simulink subsystem "PowerSystemRefAeronomie"  (R2024b)
settings: Solver=VariableStepAuto  StartTime=0.0  StopTime=10.0  RelTol=1e-3
undefined symbols (not defined in the file or in its folder): ess, mot, powerplant, propel, pxf_diagram_options, SimIn, tc
libraries: simulink x2, slpidlib x1, matrix_library x1
(part 3 of 3)

== system PowerSystemRefAeronomie/ess (battery)/ctrl/ess_ctrl_pngv_map_anl_PI_cstr/PI controller for maximal charge power and current1/PI Ratio Calculator (curr) 1 ==
  note: %deviation
  ess pwr : Inport
  pwr max cont : Inport  Port=2
  Add1 : Sum  Inputs=-+
  Integrator1 : Integrator  InitialCondition=ess.plant.init.ul_curr_dis  LimitOutput=on  UpperSaturationLimit=ess.plant.init.ul_curr_dis  LowerSaturationLimit=ess.plant.init.ll_curr_dis
  Ki_pwr : Gain  Gain=ess.plant.init.Ki_pwr_chg  SaturateOnIntegerOverflow=on  OutDataTypeStr=Inherit: Same as input  ParamDataTypeStr=Inherit: Same as input
  Saturation1 : Saturate  UpperLimit=1  LowerLimit=0
  non-zero division1 : Subsystem
      mask Display: disp('divider')
  pwr ratio : Outport
  wires:
  Add1/1 -> non-zero division1/1(In1)
  non-zero division1/1(Out1) -> Ki_pwr/1
  Ki_pwr/1 -> Integrator1/1
  Integrator1/1 -> Saturation1/1
  ess pwr/1 -> Add1/1
  Saturation1/1 -> pwr ratio/1
  pwr max cont/1 -> Add1/2, non-zero division1/2(In2)

== system PowerSystemRefAeronomie/ess (battery)/ctrl/ess_ctrl_pngv_map_anl_PI_cstr/PI controller for maximal discharge power and current1/PI Ratio Calculator (curr)  ==
  note: %deviation
  ess curr : Inport
  curr max cont : Inport  Port=2
  Add1 : Sum  Inputs=-+
  Integrator1 : Integrator  InitialCondition=ess.plant.init.ul_curr_dis  LimitOutput=on  UpperSaturationLimit=ess.plant.init.ul_curr_dis  LowerSaturationLimit=ess.plant.init.ll_curr_dis
  Ki_curr : Gain  Gain=ess.plant.init.Ki_curr_dis  SaturateOnIntegerOverflow=on  OutDataTypeStr=Inherit: Same as input  ParamDataTypeStr=Inherit: Same as input
  Saturation1 : Saturate  UpperLimit=1  LowerLimit=0
  non-zero division1 : Subsystem
      mask Display: disp('divider')
  Current ratio : Outport
  wires:
  curr max cont/1 -> non-zero division1/2(In2), Add1/2
  Saturation1/1 -> Current ratio/1
  ess curr/1 -> Add1/1
  Integrator1/1 -> Saturation1/1
  Ki_curr/1 -> Integrator1/1
  non-zero division1/1(Out1) -> Ki_curr/1
  Add1/1 -> non-zero division1/1(In1)

== system PowerSystemRefAeronomie/ess (battery)/ctrl/ess_ctrl_pngv_map_anl_PI_cstr/PI controller for maximal discharge power and current1/PI Ratio Calculator (curr) 1 ==
  note: %deviation
  ess pwr : Inport
  pwr max cont : Inport  Port=2
  Add1 : Sum  Inputs=-+
  Integrator1 : Integrator  InitialCondition=ess.plant.init.ul_curr_dis  LimitOutput=on  UpperSaturationLimit=ess.plant.init.ul_curr_dis  LowerSaturationLimit=ess.plant.init.ll_curr_dis
  Ki_pwr : Gain  Gain=ess.plant.init.Ki_pwr_dis  SaturateOnIntegerOverflow=on  OutDataTypeStr=Inherit: Same as input  ParamDataTypeStr=Inherit: Same as input
  Saturation1 : Saturate  UpperLimit=1  LowerLimit=0
  non-zero division1 : Subsystem
      mask Display: disp('divider')
  pwr ratio : Outport
  wires:
  Add1/1 -> non-zero division1/1(In1)
  non-zero division1/1(Out1) -> Ki_pwr/1
  Ki_pwr/1 -> Integrator1/1
  Integrator1/1 -> Saturation1/1
  ess pwr/1 -> Add1/1
  Saturation1/1 -> pwr ratio/1
  pwr max cont/1 -> Add1/2, non-zero division1/2(In2)

== system PowerSystemRefAeronomie/ess (battery)/plant/ess_plant_pngv_map_anl_PI_cstr/ess_cell/current polarization ==
  ess soc : Inport
  ess curr : Inport  Port=2
  Integrator : Integrator
  Product1 : Product  Inputs=*/  InputSameDT=on  SaturateOnIntegerOverflow=on  OutDataTypeStr=Inherit: Same as first input
  Sum1 : Sum  Inputs=+-  InputSameDT=on  SaturateOnIntegerOverflow=on  OutDataTypeStr=Inherit: Same as first input
  Time Constant : Lookup  InputValues=ess.plant.init.tau1.idx1_soc  Table=ess.plant.init.tau1.map
  ess_cell_curr_polar1 : Outport
  wires:
  Time Constant/1 -> Product1/2
  Product1/1 -> Integrator/1
  ess soc/1 -> Time Constant/1
  ess curr/1 -> Sum1/1
  Sum1/1 -> Product1/1
  Integrator/1 -> Sum1/2, ess_cell_curr_polar1/1

== system PowerSystemRefAeronomie/ess (battery)/plant/ess_plant_pngv_map_anl_PI_cstr/ess_cell/current polarization1 ==
  ess soc : Inport
  ess curr : Inport  Port=2
  Integrator : Integrator
  Product1 : Product  Inputs=*/  InputSameDT=on  SaturateOnIntegerOverflow=on  OutDataTypeStr=Inherit: Same as first input
  Sum1 : Sum  Inputs=+-  InputSameDT=on  SaturateOnIntegerOverflow=on  OutDataTypeStr=Inherit: Same as first input
  Time Constant : Lookup  InputValues=ess.plant.init.tau2.idx1_soc  Table=ess.plant.init.tau2.map
  ess_cell_curr_polar2 : Outport
  wires:
  Integrator/1 -> ess_cell_curr_polar2/1, Sum1/2
  Sum1/1 -> Product1/1
  ess curr/1 -> Sum1/1
  ess soc/1 -> Time Constant/1
  Product1/1 -> Integrator/1
  Time Constant/1 -> Product1/2

== system PowerSystemRefAeronomie/ess (battery)/plant/ess_plant_pngv_map_anl_PI_cstr/ess_cell/ess_soc_calculation ==
  cell_curr : Inport
  (sec->hrs) : Gain  Gain=1/3600  SaturateOnIntegerOverflow=on  OutDataTypeStr=Inherit: Same as input  ParamDataTypeStr=Inherit: Same as input
  (sec->hrs)1 : Gain  Gain=-1  SaturateOnIntegerOverflow=on  OutDataTypeStr=Inherit: Same as input  ParamDataTypeStr=Inherit: Same as input
  0 <= SOC <= 1 : Saturate  UpperLimit=1  LowerLimit=0
  1\ess.plant.init.cap : Gain  Gain=1/ess.plant.init.cap  SaturateOnIntegerOverflow=on  OutDataTypeStr=Inherit: Same as input  ParamDataTypeStr=Inherit: Same as input
  Integrator : Integrator  InitialCondition=ess.plant.init.soc_init
  ess_soc : Outport
  wires:
  (sec->hrs)/1 -> 1\ess.plant.init.cap/1
  0 <= SOC <= 1/1 -> ess_soc/1
  Integrator/1 -> 0 <= SOC <= 1/1
  (sec->hrs)1/1 -> Integrator/1
  1\ess.plant.init.cap/1 -> (sec->hrs)1/1
  cell_curr/1 -> (sec->hrs)/1

== system PowerSystemRefAeronomie/ess (battery)/plant/ess_plant_pngv_map_anl_PI_cstr/ess_cell/voltage calculation ==
  absolute SOC : Inport
  ess_cell_curr : Inport  Port=2
  ess_cell_curr_pol1 : Inport  Port=3
  ess_cell_curr_plo2 : Inport  Port=4
  Ohmic resist : Lookup  InputValues=ess.plant.init.rint.idx1_soc  Table=ess.plant.init.rint.map
  "Polarization resist 2 " : Lookup  InputValues=ess.plant.init.rpol2.idx1_soc  Table=ess.plant.init.rpol2.map
  Polarization resist2 : Lookup  InputValues=ess.plant.init.rpol1.idx1_soc  Table=ess.plant.init.rpol1.map
  Product1 : Product  InputSameDT=on  SaturateOnIntegerOverflow=on  OutDataTypeStr=Inherit: Same as first input
  Product2 : Product  InputSameDT=on  SaturateOnIntegerOverflow=on  OutDataTypeStr=Inherit: Same as first input
  Product3 : Product  InputSameDT=on  SaturateOnIntegerOverflow=on  OutDataTypeStr=Inherit: Same as first input
  Saturation : Saturate  UpperLimit=inf  LowerLimit=ess.plant.init.volt_min_burst
  Sum2 : Sum  Inputs=+---  InputSameDT=on  SaturateOnIntegerOverflow=on  OutDataTypeStr=Inherit: Same as first input
  Voc : Lookup  InputValues=ess.plant.init.voc.idx1_soc  Table=ess.plant.init.voc.map
  ess_cell_volt : Outport
  ess_cell_voc : Outport  Port=2
  ess_cell_rint : Outport  Port=3
  ess_cell_rpol1 : Outport  Port=4
  ess_cell_rpol2 : Outport  Port=5
  wires:
  Saturation/1 -> ess_cell_volt/1
  "Polarization resist 2 "/1 -> ess_cell_rpol2/1, Product3/2  "ess_rpol2_simu"
  ess_cell_curr_plo2/1 -> Product3/1
  Product3/1 -> Sum2/4
  Product2/1 -> Sum2/3
  Polarization resist2/1 -> ess_cell_rpol1/1, Product2/2  "ess_rpol1_simu"
  ess_cell_curr_pol1/1 -> Product2/1
  Product1/1 -> Sum2/2
  absolute SOC/1 -> Voc/1, Ohmic resist/1, Polarization resist2/1, "Polarization resist 2 "/1
  Voc/1 -> ess_cell_voc/1, Sum2/1  "ess_voc_simu"
  ess_cell_curr/1 -> Product1/1
  Ohmic resist/1 -> ess_cell_rint/1, Product1/2  "ess_rint_simu"
  Sum2/1 -> Saturation/1

== system PowerSystemRefAeronomie/mot/ctrl/cmd/mot_ctrl_cmd_map_Pelec_funTW_volt_in/Subsystem2 ==
  In1 : Inport
  In2 : Inport  Port=2
  Fcn : Fcn  Expr=u[1]/(u[2]+eps)*(u[2]!=0)
  Mux : Mux  Inputs=2
  Out1 : Outport
  wires:
  In2/1 -> Mux/2
  Fcn/1 -> Out1/1
  In1/1 -> Mux/1
  Mux/1 -> Fcn/1

== system PowerSystemRefAeronomie/mot/ctrl/cmd/mot_ctrl_cmd_map_Pelec_funTW_volt_in/avoid zero output ==
  In1 : Inport
  Constant : Constant  Value=eps
  Switch1 : Switch  Criteria=u2 ~= 0  SaturateOnIntegerOverflow=off  InputSameDT=off
  Out1 : Outport
  wires:
  In1/1 -> Switch1/2, Switch1/1
  Constant/1 -> Switch1/3
  Switch1/1 -> Out1/1

== system PowerSystemRefAeronomie/mot/ctrl/cstr/mot_ctrl_cstr_map_Pelec_funTW_volt_in/Continuous torque - Prop ==
  input x : Inport
  map : Lookup  InputValues=x  Table=map
  map limits on x : Saturate  UpperLimit=max(x)  LowerLimit=min(x)
  output : Outport
  wires:
  map limits on x/1 -> map/1
  map/1 -> output/1
  input x/1 -> map limits on x/1

== system PowerSystemRefAeronomie/mot/ctrl/cstr/mot_ctrl_cstr_map_Pelec_funTW_volt_in/Continuous torque _regen ==
  input x : Inport
  map : Lookup  InputValues=x  Table=map
  map limits on x : Saturate  UpperLimit=max(x)  LowerLimit=min(x)
  output : Outport
  wires:
  map limits on x/1 -> map/1
  map/1 -> output/1
  input x/1 -> map limits on x/1

== system PowerSystemRefAeronomie/mot/ctrl/cstr/mot_ctrl_cstr_map_Pelec_funTW_volt_in/Peak torque - Prop ==
  input x : Inport
  map : Lookup  InputValues=x  Table=map
  map limits on x : Saturate  UpperLimit=max(x)  LowerLimit=min(x)
  output : Outport
  wires:
  map limits on x/1 -> map/1
  map/1 -> output/1
  input x/1 -> map limits on x/1

== system PowerSystemRefAeronomie/mot/ctrl/cstr/mot_ctrl_cstr_map_Pelec_funTW_volt_in/Peak torque _regen ==
  input x : Inport
  map : Lookup  InputValues=x  Table=map
  map limits on x : Saturate  UpperLimit=max(x)  LowerLimit=min(x)
  output : Outport
  wires:
  map limits on x/1 -> map/1
  map/1 -> output/1
  input x/1 -> map limits on x/1

== system PowerSystemRefAeronomie/mot/ctrl/dmd/mot_ctrl_dmd_uas/Determine_Required_Motor_RPS ==
  Prop_D : Inport
  rho : Inport  Port=2
  P : Inport  Port=3
  Vtas : Inport  Port=4
  Algebraic Constraint1 : AlgebraicConstraint  InitialGuess=propel.ctrl.init.rps
  CP : Polyval  Coefs=powerplant.propel.init.CPpoly
  Fcn1 : Fcn  Expr=u(4)*u(5)^3 - u(3)/(u(2)*u(1)^5)
  Mux1 : Mux  Inputs=5
  Product : Product  Inputs=*//
  RPS_req : Outport  VectorParamsAs1DForOutWhenUnconnected=off
  wires:
  Vtas/1 -> Product/1
  Prop_D/1 -> Mux1/1, Product/2
  CP/1 -> Mux1/4
  Product/1 -> CP/1
  P/1 -> Mux1/3
  Mux1/1 -> Fcn1/1
  Fcn1/1 -> Algebraic Constraint1/1
  Algebraic Constraint1/1 -> RPS_req/1, Mux1/5, Product/3  "RPS_req"
  rho/1 -> Mux1/2

== system PowerSystemRefAeronomie/mot/ctrl/dmd/parameter_selection/Subsystem ==
  <EngineCmd> : Inport
  <Density> : Inport  Port=2
  Vtas : Inport  Port=3
  CP : Polyval  Coefs=powerplant.propel.init.CPpoly
  Constant8 : Constant  Value=mot.propel.plant.init.propD
  Fcn : Fcn  Expr=u(1)*u(2)*u(3)^3*u(4)^5
  Mux : Mux
  Normalize : Gain  Gain=1/mot.propel.plant.init.Pmax
  Product : Product  Inputs=*//
  Selector : Selector  InputPortWidth=9  IndexOptions=Index vector (dialog)  Indices=9  OutputSizes=1
  Transfer Fcn : TransferFcn  Numerator=1  Denominator=[0.01 1]
  rad/s to RPS : Gain  Gain=1/(2*pi)
  EnginePwrCmd : Outport
  wires:
  Fcn/1 -> Normalize/1
  Transfer Fcn/1 -> EnginePwrCmd/1
  rad/s to RPS/1 -> Mux/3, Product/3
  Vtas/1 -> Product/1
  Normalize/1 -> Transfer Fcn/1
  Mux/1 -> Fcn/1
  Selector/1 -> rad/s to RPS/1
  <Density>/1 -> Mux/2
  CP/1 -> Mux/1
  <EngineCmd>/1 -> Selector/1
  Constant8/1 -> Mux/4, Product/2
  Product/1 -> CP/1

== system PowerSystemRefAeronomie/mot/plant/mot_plant_map_Pelec_funTW_volt_in/max torque /Cont trq max - Prop ==
  input x : Inport
  map : Lookup  InputValues=x  Table=map
  map limits on x : Saturate  UpperLimit=max(x)  LowerLimit=min(x)
  output : Outport
  wires:
  input x/1 -> map limits on x/1
  map/1 -> output/1
  map limits on x/1 -> map/1

== system PowerSystemRefAeronomie/mot/plant/mot_plant_map_Pelec_funTW_volt_in/max torque /Cont trq max - Regen ==
  input x : Inport
  map : Lookup  InputValues=x  Table=map
  map limits on x : Saturate  UpperLimit=max(x)  LowerLimit=min(x)
  output : Outport
  wires:
  map limits on x/1 -> map/1
  map/1 -> output/1
  input x/1 -> map limits on x/1

== system PowerSystemRefAeronomie/mot/plant/mot_plant_map_Pelec_funTW_volt_in/max torque /Heat index ==
  note: Heat index calculation
  note: to avoid spikes
      |  due to
      | div by zero
  cont torque : Inport
  torque : Inport  Port=2
  Abs : Abs
  Divide : Subsystem  mask(Divide){}
      mask Display: disp('Divide')
  Heat Energy Factor : Integrator  InitialCondition=-0.3  LimitOutput=on  UpperSaturationLimit=1  LowerSaturationLimit=-0.3
  Heating Constant : Gain  Gain=0.3/mot.plant.init.t_max_trq  SaturateOnIntegerOverflow=on  OutDataTypeStr=Inherit: Same as input  ParamDataTypeStr=Inherit: Same as input
  Saturation : Saturate  UpperLimit=1  LowerLimit=0
  Saturation1 : Saturate  UpperLimit=10  LowerLimit=0
  Sum : Sum  Inputs=+-  InputSameDT=on  SaturateOnIntegerOverflow=on  OutDataTypeStr=Inherit: Same as first input
  motor inertia (Nms^2\rad)5 : Constant
  Heat index : Outport
  wires:
  Saturation1/1 -> Sum/1
  torque/1 -> Divide/1(numerator)
  Heat Energy Factor/1 -> Saturation/1
  Heating Constant/1 -> Heat Energy Factor/1
  Sum/1 -> Heating Constant/1
  Divide/1(quotient) -> Abs/1
  motor inertia (Nms^2\rad)5/1 -> Sum/2
  Saturation/1 -> Heat index/1
  Abs/1 -> Saturation1/1
  cont torque/1 -> Divide/2(denominator)

== system PowerSystemRefAeronomie/mot/plant/mot_plant_map_Pelec_funTW_volt_in/max torque /Peak trq max - Prop ==
  input x : Inport
  map : Lookup  InputValues=x  Table=map
  map limits on x : Saturate  UpperLimit=max(x)  LowerLimit=min(x)
  output : Outport
  wires:
  map limits on x/1 -> map/1
  map/1 -> output/1
  input x/1 -> map limits on x/1

== system PowerSystemRefAeronomie/mot/plant/mot_plant_map_Pelec_funTW_volt_in/max torque /Peak trq max - Regen ==
  input x : Inport
  map : Lookup  InputValues=x  Table=map
  map limits on x : Saturate  UpperLimit=max(x)  LowerLimit=min(x)
  output : Outport
  wires:
  input x/1 -> map limits on x/1
  map/1 -> output/1
  map limits on x/1 -> map/1

== system PowerSystemRefAeronomie/propel/plant/propel_plant_uas/Total_Moment/Moment_due_to_eng_position ==
  Vec 1 : Inport
  Vec 2 : Inport  Port=2
  Mux : Mux  Inputs=2
  Mux1 : Mux  Inputs=3
  i axis : Fcn  Expr=u[6]*u[2] - u[5]*u[3]
  j axis : Fcn  Expr=u[4]*u[3] - u[6]*u[1]
  k axis : Fcn  Expr=u[5]*u[1] - u[4]*u[2]
  X Prod : Outport  VectorParamsAs1DForOutWhenUnconnected=off
  wires:
  Mux1/1 -> X Prod/1
  k axis/1 -> Mux1/3
  i axis/1 -> Mux1/1
  j axis/1 -> Mux1/2
  Mux/1 -> i axis/1, k axis/1, j axis/1
  Vec 1/1 -> Mux/1
  Vec 2/1 -> Mux/2

== system PowerSystemRefAeronomie/tc/plant/tc_plant_map_trqloss_funTW/Torque calculation/Blending (state dependent) ==
  Input : Inport
  Control (state) : Inport  Port=2
  Linear spline : Fcn  Expr=(u<xl)*yl + (xl<=u)*(u<xc)*((yc-yl)*(u-xl)/(xc-xl)+yl) + (xc<=u)*(u<xr)*((yc-yr)*(u-xr)/(xc-xr)+yr) + (xr<=u)*yr
  Product2 : Product  InputSameDT=on  SaturateOnIntegerOverflow=on  OutDataTypeStr=Inherit: Same as first input
  Output : Outport
  wires:
  Input/1 -> Product2/1
  Linear spline/1 -> Product2/2
  Product2/1 -> Output/1
  Control (state)/1 -> Linear spline/1

== system PowerSystemRefAeronomie/tc/plant/tc_plant_map_trqloss_funTW/Torque calculation/trq losses ==
  Rows : Inport
  Cols : Inport  Port=2
  Look-Up Table (2-D) : Lookup2D  RowIndex=x  ColumnIndex=y  Table=t
  Out1 : Outport
  wires:
  Look-Up Table (2-D)/1 -> Out1/1
  Cols/1 -> Look-Up Table (2-D)/2
  Rows/1 -> Look-Up Table (2-D)/1

== system PowerSystemRefAeronomie/ess (battery)/ctrl/ess_ctrl_pngv_map_anl_PI_cstr/PI controller for maximal charge power and current1/PI Ratio Calculator (curr) /non-zero division1 ==
  note: original idea from Phil Sharer - ANL
      | original formula: u[1]\(u[2]+eps)*(u[2]!=0)
      | changes done by Gerald ZINI (dgey) - ANL (05\02\2001)
  note: (u[2]==0) is true then returns 1, thus (u[2]+(u[2]==0)) is equal to 0+1=1
  note: if u[2] == 0, then output == 0:
  note: (u[2]!=0) is false then returns 0
  note: and finally, the expression is: (u[1] \ 1) * 0 = 0
  note: (u[2]==0) is false then returns 0, thus (u[2]+(u[2]==0)) is equal to u[2]+0=u[2]
  note: if u[2] != 0, then output == u[1]\u[2]:
  note: (u[2]!=0) is true then returns 1
  note: and finally, the expression is: (u[1] \ u[2]) * 1 = u[1] \ u[2]
  In1 : Inport
  In2 : Inport  Port=2
  Fcn : Fcn  Expr=u[1]/(u[2]+(u[2]==0))*(u[2]!=0)
  Mux : Mux  Inputs=2
  Out1 : Outport
  wires:
  Mux/1 -> Fcn/1
  In1/1 -> Mux/1
  Fcn/1 -> Out1/1
  In2/1 -> Mux/2

== system PowerSystemRefAeronomie/ess (battery)/ctrl/ess_ctrl_pngv_map_anl_PI_cstr/PI controller for maximal charge power and current1/PI Ratio Calculator (curr) 1/non-zero division1 ==
  note: original idea from Phil Sharer - ANL
      | original formula: u[1]\(u[2]+eps)*(u[2]!=0)
      | changes done by Gerald ZINI (dgey) - ANL (05\02\2001)
  note: (u[2]==0) is true then returns 1, thus (u[2]+(u[2]==0)) is equal to 0+1=1
  note: if u[2] == 0, then output == 0:
  note: (u[2]!=0) is false then returns 0
  note: and finally, the expression is: (u[1] \ 1) * 0 = 0
  note: (u[2]==0) is false then returns 0, thus (u[2]+(u[2]==0)) is equal to u[2]+0=u[2]
  note: if u[2] != 0, then output == u[1]\u[2]:
  note: (u[2]!=0) is true then returns 1
  note: and finally, the expression is: (u[1] \ u[2]) * 1 = u[1] \ u[2]
  In1 : Inport
  In2 : Inport  Port=2
  Fcn : Fcn  Expr=u[1]/(u[2]+(u[2]==0))*(u[2]!=0)
  Mux : Mux  Inputs=2
  Out1 : Outport
  wires:
  Mux/1 -> Fcn/1
  In1/1 -> Mux/1
  Fcn/1 -> Out1/1
  In2/1 -> Mux/2

== system PowerSystemRefAeronomie/ess (battery)/ctrl/ess_ctrl_pngv_map_anl_PI_cstr/PI controller for maximal discharge power and current1/PI Ratio Calculator (curr) /non-zero division1 ==
  note: and finally, the expression is: (u[1] \ u[2]) * 1 = u[1] \ u[2]
  note: (u[2]!=0) is true then returns 1
  note: if u[2] != 0, then output == u[1]\u[2]:
  note: (u[2]==0) is false then returns 0, thus (u[2]+(u[2]==0)) is equal to u[2]+0=u[2]
  note: and finally, the expression is: (u[1] \ 1) * 0 = 0
  note: (u[2]!=0) is false then returns 0
  note: if u[2] == 0, then output == 0:
  note: (u[2]==0) is true then returns 1, thus (u[2]+(u[2]==0)) is equal to 0+1=1
  note: original idea from Phil Sharer - ANL
      | original formula: u[1]\(u[2]+eps)*(u[2]!=0)
      | changes done by Gerald ZINI (dgey) - ANL (05\02\2001)
  In1 : Inport
  In2 : Inport  Port=2
  Fcn : Fcn  Expr=u[1]/(u[2]+(u[2]==0))*(u[2]!=0)
  Mux : Mux  Inputs=2
  Out1 : Outport
  wires:
  In2/1 -> Mux/2
  Fcn/1 -> Out1/1
  In1/1 -> Mux/1
  Mux/1 -> Fcn/1

== system PowerSystemRefAeronomie/ess (battery)/ctrl/ess_ctrl_pngv_map_anl_PI_cstr/PI controller for maximal discharge power and current1/PI Ratio Calculator (curr) 1/non-zero division1 ==
  note: original idea from Phil Sharer - ANL
      | original formula: u[1]\(u[2]+eps)*(u[2]!=0)
      | changes done by Gerald ZINI (dgey) - ANL (05\02\2001)
  note: (u[2]==0) is true then returns 1, thus (u[2]+(u[2]==0)) is equal to 0+1=1
  note: if u[2] == 0, then output == 0:
  note: (u[2]!=0) is false then returns 0
  note: and finally, the expression is: (u[1] \ 1) * 0 = 0
  note: (u[2]==0) is false then returns 0, thus (u[2]+(u[2]==0)) is equal to u[2]+0=u[2]
  note: if u[2] != 0, then output == u[1]\u[2]:
  note: (u[2]!=0) is true then returns 1
  note: and finally, the expression is: (u[1] \ u[2]) * 1 = u[1] \ u[2]
  In1 : Inport
  In2 : Inport  Port=2
  Fcn : Fcn  Expr=u[1]/(u[2]+(u[2]==0))*(u[2]!=0)
  Mux : Mux  Inputs=2
  Out1 : Outport
  wires:
  Mux/1 -> Fcn/1
  In1/1 -> Mux/1
  Fcn/1 -> Out1/1
  In2/1 -> Mux/2

== system PowerSystemRefAeronomie/mot/plant/mot_plant_map_Pelec_funTW_volt_in/max torque /Heat index/Divide ==
  note: Take care of
      | division by 0
  numerator : Inport
  denominator : Inport  Port=2
  Fcn : Fcn  Expr=u[1] / ( u[2] + eps*(u[2]==0) )
  Mux : Mux  Inputs=2
  quotient : Outport
  wires:
  Mux/1 -> Fcn/1
  numerator/1 -> Mux/1
  Fcn/1 -> quotient/1
  denominator/1 -> Mux/2
